simulink model "Middle_speed_sim"  (R2016a)
settings: Solver=VariableStepAuto  StartTime=0.0  StopTime=100  RelTol=1e-3
values from neighbouring files (symbols this model uses):
  Kp2 = cp2*wL    (= 12)    [Middle_speed.m]
  Kv2 = cv2*wL    (= 48)    [Middle_speed.m]
libraries: simulink x1
settings Model: Creator=DELL  LastModifiedBy=DELL

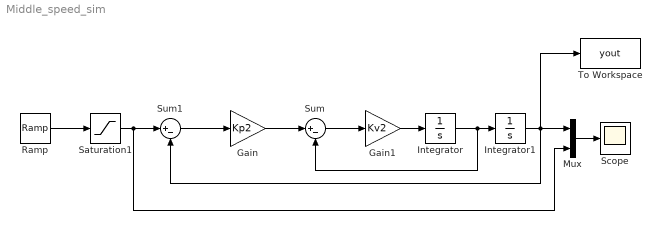
== system Middle_speed_sim ==
  Gain : Gain  Gain=Kp2
  Gain1 : Gain  Gain=Kv2
  Integrator : Integrator
  Integrator1 : Integrator
  Mux : Mux  Inputs=2
  Ramp : simulink/Sources/Ramp  slope=1  start=0  X0=0
  Saturation1 : Saturate  UpperLimit=10  LowerLimit=0
  Scope : Scope
  Sum : Sum  Inputs=|+-
  Sum1 : Sum  Inputs=|+-
  To Workspace : ToWorkspace  VariableName=yout  SaveFormat=Timeseries  SampleTime=-1
  wires:
  Sum1/1 -> Gain/1
  Ramp/1 -> Saturation1/1
  Gain/1 -> Sum/1
  Sum/1 -> Gain1/1
  Gain1/1 -> Integrator/1
  Integrator/1 -> Sum/2, Integrator1/1
  Saturation1/1 -> Mux/2, Sum1/1
  Mux/1 -> Scope/1
  Integrator1/1 -> To Workspace/1, Sum1/2, Mux/1
